simulink model "DC_Motor_Control_SPS_rectifier"  (R2024a)
settings: Solver=VariableStepAuto  StartTime=0.0  StopTime=20  RelTol=1e-3
undefined symbols (not defined in the file): D1, Kd_i, Ki_i, Ki_w, Kp_i, Kp_w, lagging, pulse
libraries: slpidlib x2, spsCurrentMeasurementLib x1, spsDCMachineLib x1, spsPulseGeneratorThyristor6PulseLib x1, spsSeriesRLCBranchLib x1, spsThreePhaseSourceLib x1, spsUniversalBridgeLib x1, spsVoltageMeasurementLib x1, spspowerguiLib x1
settings Model: Creator=Lagha  LastModifiedBy=Administrator

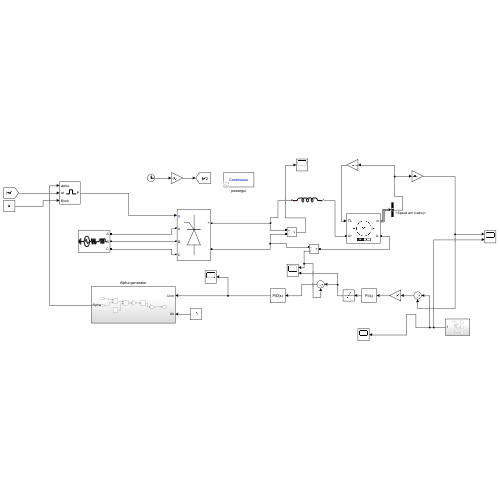
[thumbnail: Simulink's stored preview of the top-level diagram]
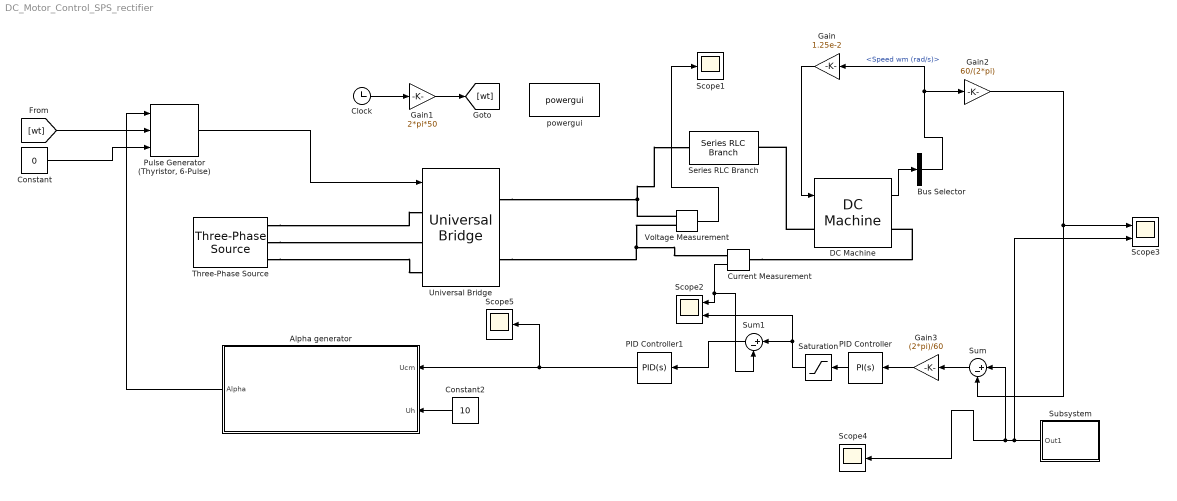
== system DC_Motor_Control_SPS_rectifier ==
  Alpha generator : Subsystem
  Bus Selector : BusSelector  OutputSignals=Speed wm (rad/s)
  Clock : Clock
  Constant : Constant  Value=0
  Constant2 : Constant  Value=10
  Current Measurement : spsCurrentMeasurementLib/Current Measurement  PhasorSimulation=off  OutputType=Complex  PSBequivalent=0
  DC Machine : spsDCMachineLib/DC Machine  PresetModel=No  MechanicalLoad=Torque TL  FieldType=Permanent magnet  ShowDetailedParameters=on  MeasurementBus=off  RLa="[ 2.33  0.0106]"  RLf="[ 240  120]"  Laf=1.8  MachineConstant=Torque constant (N.m/A)  Ke=1.8  Kt=0.57  J=7.5e-3  Bm=1.75e-4  Tf=0  w0=0  Ifinit=1  TsPowergui=0  TsBlock=-1
  Gain : Gain  Gain=1.25e-2
  Gain1 : Gain  Gain=2*pi*50
  Gain2 : Gain  Gain=60/(2*pi)
  Gain3 : Gain  Gain=(2*pi)/60
  PID Controller : slpidlib/PID Controller  Controller=PI  Form=Parallel  TimeDomain=Continuous-time  UseExternalTs=off  SampleTime=-1  IntegratorMethod=Forward Euler  FilterMethod=Forward Euler  ControllerParametersSource=internal  P=Kp_w  I=Ki_w  UseKiTs=off  D=0  UseExternalDerivativeSource=off  N=100  UseFilter=on  TunerSelectOption=Transfer Function Based (PID Tuner App)  InitialConditionSource=internal  InitialConditionForIntegrator=0  InitialConditionForFilter=0  DifferentiatorICPrevScaledInput=0  ExternalReset=none  TrackingMode=off  Kt=1  LimitOutput=off  SatLimitsSource=internal  UpperSaturationLimit=inf  LowerSaturationLimit=-inf  LinearizeAsGain=on  AntiWindupMode=none  Kb=1  LimitIntegrator=off  UpperIntegratorSaturationLimit=inf  LowerIntegratorSaturationLimit=-inf  POutMin=[]  POutMax=[]  IOutMin=[]  IOutMax=[]  DOutMin=[]  DOutMax=[]  NOutMin=[]  NOutMax=[]  SumOutMin=[]  SumOutMax=[]  SaturationOutMin=[]  SaturationOutMax=[]  PParamMin=[]  PParamMax=[]  IParamMin=[]  IParamMax=[]  DParamMin=[]  DParamMax=[]  NParamMin=[]  NParamMax=[]  KbParamMin=[]  KbParamMax=[]  KtParamMin=[]  KtParamMax=[]  KbOutMin=[]  KbOutMax=[]  KtOutMin=[]  KtOutMax=[]  IntegratorOutMin=[]  IntegratorOutMax=[]  FilterOutMin=[]  FilterOutMax=[]  SumI1OutMin=[]  SumI1OutMax=[]  SumI2OutMin=[]  SumI2OutMax=[]  SumI3OutMin=[]  SumI3OutMax=[]  SumI4OutMin=[]  SumI4OutMax=[]  SumDOutMin=[]  SumDOutMax=[]  DifferentiatorOutMin=[]  DifferentiatorOutMax=[]  FilterDiffOutCoefMin=[]  FilterDiffOutCoefMax=[]  ReciprocalOutMin=[]  ReciprocalOutMax=[]  SumDenOutMin=[]  SumDenOutMax=[]  SumNumOutMin=[]  SumNumOutMax=[]  DivideOutMin=[]  DivideOutMax=[]  UdiffTsProdOutMin=[]  UdiffTsProdOutMax=[]  NTsProdOutMin=[]  NTsProdOutMax=[]  UintegralTsProdOutMin=[]  UintegralTsProdOutMax=[]  UngainTsProdOutMin=[]  UngainTsProdOutMax=[]  ClampingZeroOutDataTypeStr=Inherit: Inherit via back propagation  ClampingZeroOutMin=[]  ClampingZeroOutMax=[]  FilterDenConstantOutDataTypeStr=Inherit: Inherit via back propagation  FilterDenConstantOutMin=[]  FilterDenConstantOutMax=[]  PCopyOutDataTypeStr=Inherit: Inherit via back propagation  PCopyOutMin=[]  PCopyOutMax=[]  NCopyOutDataTypeStr=Inherit: Inherit via back propagation  NCopyOutMin=[]  NCopyOutMax=[]  IntegratorContinuousStateAttributes=''  IntegratorStateMustResolveToSignalObject=off  IntegratorRTWStateStorageClass=Auto  FilterContinuousStateAttributes=''  FilterStateMustResolveToSignalObject=off  FilterRTWStateStorageClass=Auto  ParallelPVariant=InternalParameters  IdealPVariant=Disabled  IVariant=InternalParameters  DVariant=Disabled  IntegratorVariant=Continuous  SatVariant=Disabled  AWVariant=Passthrough  PCopyVariant=Disabled  TRVariant=Disabled  FdbkBlocksVariant=Forward  IdealPFdbkVariant=Disabled  SatFdbkVariant=Disabled  DerivativeFilterVariant=Disabled  NVariant=Disabled  NCopyVariant=Disabled_SignalSpec  FilterICVariant=Disabled  IntegratorICVariant=InternalICs  ExternalResetVariant=Disabled  TRSumVariant=Passthrough  SumFdbkVariant=Disabled  SumVariant=Sum_PI  TsampFilterVariant=InternalTs  TsampNgainVariant=Passthrough  TsampIntegralVariant=Disabled_SignalSpec  ExternalSaturationOutDataTypeStr=Inherit: Same as second input  DerivativeSourceVariant=Disabled
  PID Controller1 : slpidlib/PID Controller  Controller=PID  Form=Parallel  TimeDomain=Continuous-time  UseExternalTs=off  SampleTime=-1  IntegratorMethod=Forward Euler  FilterMethod=Forward Euler  ControllerParametersSource=internal  P=Kp_i  I=Ki_i  UseKiTs=off  D=Kd_i  UseExternalDerivativeSource=off  N=100  UseFilter=on  TunerSelectOption=Transfer Function Based (PID Tuner App)  InitialConditionSource=internal  InitialConditionForIntegrator=0  InitialConditionForFilter=0  DifferentiatorICPrevScaledInput=0  ExternalReset=none  TrackingMode=off  Kt=1  LimitOutput=off  SatLimitsSource=internal  UpperSaturationLimit=inf  LowerSaturationLimit=-inf  LinearizeAsGain=on  AntiWindupMode=none  Kb=1  LimitIntegrator=off  UpperIntegratorSaturationLimit=inf  LowerIntegratorSaturationLimit=-inf  POutMin=[]  POutMax=[]  IOutMin=[]  IOutMax=[]  DOutMin=[]  DOutMax=[]  NOutMin=[]  NOutMax=[]  SumOutMin=[]  SumOutMax=[]  SaturationOutMin=[]  SaturationOutMax=[]  PParamMin=[]  PParamMax=[]  IParamMin=[]  IParamMax=[]  DParamMin=[]  DParamMax=[]  NParamMin=[]  NParamMax=[]  KbParamMin=[]  KbParamMax=[]  KtParamMin=[]  KtParamMax=[]  KbOutMin=[]  KbOutMax=[]  KtOutMin=[]  KtOutMax=[]  IntegratorOutMin=[]  IntegratorOutMax=[]  FilterOutMin=[]  FilterOutMax=[]  SumI1OutMin=[]  SumI1OutMax=[]  SumI2OutMin=[]  SumI2OutMax=[]  SumI3OutMin=[]  SumI3OutMax=[]  SumI4OutMin=[]  SumI4OutMax=[]  SumDOutMin=[]  SumDOutMax=[]  DifferentiatorOutMin=[]  DifferentiatorOutMax=[]  FilterDiffOutCoefMin=[]  FilterDiffOutCoefMax=[]  ReciprocalOutMin=[]  ReciprocalOutMax=[]  SumDenOutMin=[]  SumDenOutMax=[]  SumNumOutMin=[]  SumNumOutMax=[]  DivideOutMin=[]  DivideOutMax=[]  UdiffTsProdOutMin=[]  UdiffTsProdOutMax=[]  NTsProdOutMin=[]  NTsProdOutMax=[]  UintegralTsProdOutMin=[]  UintegralTsProdOutMax=[]  UngainTsProdOutMin=[]  UngainTsProdOutMax=[]  ClampingZeroOutDataTypeStr=Inherit: Inherit via back propagation  ClampingZeroOutMin=[]  ClampingZeroOutMax=[]  FilterDenConstantOutDataTypeStr=Inherit: Inherit via back propagation  FilterDenConstantOutMin=[]  FilterDenConstantOutMax=[]  PCopyOutDataTypeStr=Inherit: Inherit via back propagation  PCopyOutMin=[]  PCopyOutMax=[]  NCopyOutDataTypeStr=Inherit: Inherit via back propagation  NCopyOutMin=[]  NCopyOutMax=[]  IntegratorContinuousStateAttributes=''  IntegratorStateMustResolveToSignalObject=off  IntegratorRTWStateStorageClass=Auto  FilterContinuousStateAttributes=''  FilterStateMustResolveToSignalObject=off  FilterRTWStateStorageClass=Auto  ParallelPVariant=InternalParameters  IdealPVariant=Disabled  IVariant=InternalParameters  DVariant=InternalParameters  IntegratorVariant=Continuous  SatVariant=Disabled  AWVariant=Passthrough  PCopyVariant=Disabled  TRVariant=Disabled  FdbkBlocksVariant=Forward  IdealPFdbkVariant=Disabled  SatFdbkVariant=Disabled  DerivativeFilterVariant=ContFilter  NVariant=InternalParameters  NCopyVariant=Disabled  FilterICVariant=InternalICsFilter  IntegratorICVariant=InternalICs  ExternalResetVariant=Disabled  TRSumVariant=Passthrough  SumFdbkVariant=Disabled  SumVariant=Sum_PID  TsampFilterVariant=InternalTs  TsampNgainVariant=Passthrough  TsampIntegralVariant=Disabled_SignalSpec  ExternalSaturationOutDataTypeStr=Inherit: Same as second input  DerivativeSourceVariant=ErrorSignal
  "Pulse Generator (Thyristor, 6-Pulse)" : spsPulseGeneratorThyristor6PulseLib/Pulse Generator (Thyristor, 6-Pulse)  GenType=6-pulse  Delta=D1 (lagging)  pwidth=60  Double_Pulse=off  Ts=0
      settings: LibrarySourceBlock=|
      | sps_lib/Power Electronics/Power Electronics Control/Pulse Generator
      | (Thyristor, 6-Pulse)
  Saturation : Saturate  UpperLimit=7  LowerLimit=-7
  Scope1 : Scope
  Scope2 : Scope  NumInputPorts=2
  Scope3 : Scope  NumInputPorts=2
  Scope4 : Scope
  Scope5 : Scope
  Series RLC Branch : spsSeriesRLCBranchLib/Series RLC Branch  LConnTagsString=__new0  RConnTagsString=__new0  BranchType=L  Resistance=0  Inductance=276e-3  SetiL0=off  InitialCurrent=0  Capacitance=0  Setx0=off  InitialVoltage=0  Measurements=None
  Subsystem : Subsystem
  Sum : Sum  Inputs=|+-
  Sum1 : Sum  Inputs=|+-
  Three-Phase Source : spsThreePhaseSourceLib/Three-Phase Source  InternalConnection=Yg  VoltagePhases=off  Voltage=220  PhaseAngle=0  Voltage_phases=[25e3 25e3 25e3]/sqrt(3)  PhaseAngles_phases=[0 -120 +120]  Frequency=50  NonIdealSource=on  SpecifyImpedance=off  Resistance=0.8929  Inductance=16.58e-3  ShortCircuitLevel=100e6  BaseVoltage=25e3  XRratio=7  BusType=swing  Pref=10e3  Qref=0  Prefabc=[10e3, 10e3, 10e3]  Qrefabc=[0, 0, 0]  Qmin=-inf  Qmax=inf
  Universal Bridge : spsUniversalBridgeLib/Universal Bridge  Arms=3  SnubberResistance=1e5  SnubberCapacitance=inf  Device=Thyristors  Ron=1e-3  Lon=0  ForwardVoltages="[  0  0  ]"  ForwardVoltage=0  GTOparameters=[ 10e-6 , 20e-6 ]  IGBTparameters=[ 1e-6 , 2e-6 ]  Measurements=None  Measurements_2=None  converterType=Rectifier
  Voltage Measurement : spsVoltageMeasurementLib/Voltage Measurement  PhasorSimulation=off  OutputType=Complex  PSBequivalent=0
  powergui : spspowerguiLib/powergui  Priority=1  SimulationMode=Continuous  SampleTime=50e-6  frequency=50  Iterations=50  frequencyindice=0  Pbase=100e6  ErrMax=1e-4  UnitsV=kV  UnitsW=MW  buscounter=0  FunctionMessages=off  echomessages=off  EnableUseOfTLC=off  CurrentSourceSwitches=off  DisableSnubberDevices=off  DisableRonSwitches=off  DisableVfSwitches=off  DisplayEquations=off  AutomaticDiscreteSolvers=off  SolverType=Tustin/Backward Euler (TBE)  Interpol=off  ExternalGateDelay=off  methode=off  Ts=100  x0status=blocks  SPID=on  SwTol=0  HookPort=off  NonlinearTolerance=1e-4  nMaxIteration=100  ContinueOnMaxIteration=off  RestoreLinks=warning  ResistiveCurrentMeasurement=off  Frange=[0:2:500]  Ylog=off  Xlog=on  ShowGrid=off  save=off  variable=ZData  structure=0  ZoomFFT=off  StartTime=0.0  cycles=1  DisplayStyle=1  fundamental=60  FreqAxis=off  MaxFrequency=1000  frequencyindicesteady=1  RmsSteady=1  display=off
  wires:
  Voltage Measurement/1 -> Scope1/1
  Current Measurement/1 -> Sum1/2, Scope2/1
  DC Machine/1 -> Bus Selector/1
  Gain/1 -> DC Machine/1
  Bus Selector/1 -> Gain2/1, Gain/1  "<Speed wm (rad/s)>"
  Subsystem/1(Out1) -> Scope3/2, Sum/1, Scope4/1
  Sum1/1 -> PID Controller1/1
  Sum/1 -> Gain3/1
  Gain2/1 -> Sum/2, Scope3/1
  Gain3/1 -> PID Controller/1
  PID Controller/1 -> Saturation/1
  Saturation/1 -> Scope2/2, Sum1/1
  [wt] -> "Pulse Generator (Thyristor, 6-Pulse)"/2
  Alpha generator/1(Alpha) -> "Pulse Generator (Thyristor, 6-Pulse)"/1
  Constant2/1 -> Alpha generator/2(Uh)
  Constant/1 -> "Pulse Generator (Thyristor, 6-Pulse)"/3
  PID Controller1/1 -> Scope5/1, Alpha generator/1(Ucm)
  "Pulse Generator (Thyristor, 6-Pulse)"/1 -> Universal Bridge/1
  Gain1/1 -> [wt]
  Clock/1 -> Gain1/1
  connections:
  Current Measurement/LConn1 -- DC Machine/RConn1
  Voltage Measurement/LConn2 -- Universal Bridge/RConn2 -- Current Measurement/RConn1
  DC Machine/LConn1 -- Series RLC Branch/RConn1
  Voltage Measurement/LConn1 -- Universal Bridge/RConn1 -- Series RLC Branch/LConn1
  Three-Phase Source/RConn1 -- Universal Bridge/LConn1
  Three-Phase Source/RConn2 -- Universal Bridge/LConn2
  Three-Phase Source/RConn3 -- Universal Bridge/LConn3

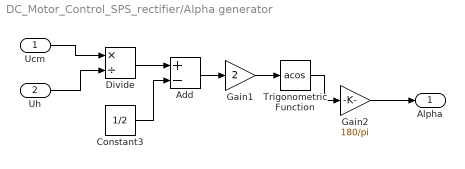
== system DC_Motor_Control_SPS_rectifier/Alpha generator ==
  Ucm : Inport
  Uh : Inport  Port=2
  Add : Sum  Inputs=+-
  Constant3 : Constant  Value=1/2
  Divide : Product  Inputs=*/
  Gain1 : Gain  Gain=2
  Gain2 : Gain  Gain=180/pi
  Trigonometric Function : Trigonometry  Operator=acos
  Alpha : Outport
  wires:
  Gain1/1 -> Trigonometric Function/1
  Uh/1 -> Divide/2
  Trigonometric Function/1 -> Gain2/1
  Gain2/1 -> Alpha/1
  Ucm/1 -> Divide/1
  Constant3/1 -> Add/2
  Divide/1 -> Add/1
  Add/1 -> Gain1/1

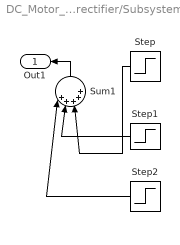
== system DC_Motor_Control_SPS_rectifier/Subsystem ==
  Step : Step  After=1000  SampleTime=0
  Step1 : Step  Time=5  After=2000  SampleTime=0
  Step2 : Step  Time=10  After=-1500  SampleTime=0
  Sum1 : Sum  Inputs=|+++++
  Out1 : Outport
  wires:
  Step1/1 -> Sum1/2
  Sum1/1 -> Out1/1
  Step2/1 -> Sum1/1
  Step/1 -> Sum1/3
